simulink model "LabPSU_CPU01"  (R2026b)
undefined symbols (not defined in the file or in its folder): bit, Ctl_ipcTs, currentMeasured, enable, measurement, openLoopSetpoint, opmode, reference, slewrate, voltageMeasured
libraries: c2802xlib x2, procinterlib x2, c2000lib x1, c2837xDlib x1
settings Model: Creator=BenjaminRupp  LastModifiedBy=BenjaminRupp

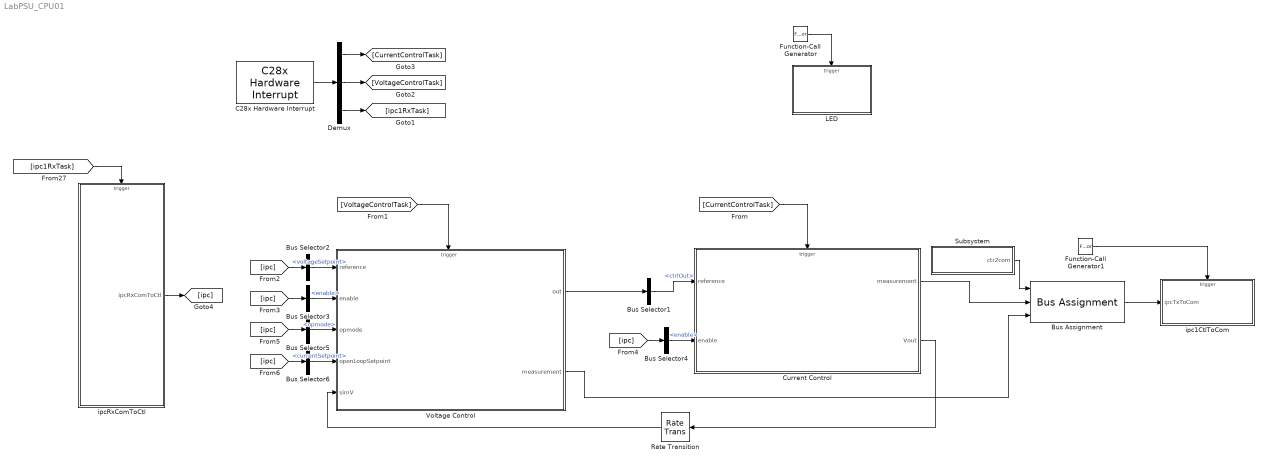
== system LabPSU_CPU01 ==
  Bus Assignment : BusAssignment  AssignedSignals=currentMeasured,voltageMeasured
  Bus Selector1 : BusSelector  OutputSignals=ctrlOut
  Bus Selector2 : BusSelector  OutputSignals=voltageSetpoint
  Bus Selector3 : BusSelector  OutputSignals=enable
  Bus Selector4 : BusSelector  OutputSignals=enable
  Bus Selector5 : BusSelector  OutputSignals=opmode
  Bus Selector6 : BusSelector  OutputSignals=currentSetpoint
  C28x Hardware Interrupt : c2000lib/Scheduling/C28x Hardware Interrupt  irqnumbers=[1 1 1]  pienumbers=[1 2 14]  irqpriorities=[30 29 28]  irqpreempts=[0 0 0]  showinput=off  dspchiptype=C280X
  Current Control : Subsystem
  Demux : Demux  Outputs=3
  Function-Call Generator : FunctionCallGenerator  SampleTime=0.1
  Function-Call Generator1 : FunctionCallGenerator  SampleTime=Ctl_ipcTs
  LED : Subsystem
  Rate Transition : RateTransition  Integrity=off
  Subsystem : Subsystem
  Voltage Control : Subsystem
  ipc1CtlToCom : Subsystem
  ipcRxComToCtl : Subsystem
  wires:
  Demux/1 -> [CurrentControlTask]
  Demux/3 -> [ipc1RxTask]
  C28x Hardware Interrupt/1 -> Demux/1
  Demux/2 -> [VoltageControlTask]
  Function-Call Generator/1 -> LED/Trigger
  [ipc1RxTask] -> ipcRxComToCtl/Trigger
  Function-Call Generator1/1 -> ipc1CtlToCom/Trigger
  [CurrentControlTask] -> Current Control/Trigger
  [VoltageControlTask] -> Voltage Control/Trigger
  Subsystem/1(ctr2com) -> Bus Assignment/1
  Bus Assignment/1 -> ipc1CtlToCom/1(ipcTxToCom)
  Current Control/1(measurement) -> Bus Assignment/2
  Voltage Control/2(measurement) -> Bus Assignment/3
  Voltage Control/1(out) -> Bus Selector1/1
  Bus Selector1/1 -> Current Control/1(reference)  "<ctrlOut>"
  ipcRxComToCtl/1(ipcRxComToCtl) -> [ipc]
  [ipc] -> Bus Selector2/1
  Bus Selector2/1 -> Voltage Control/1(reference)  "<voltageSetpoint>"
  Bus Selector3/1 -> Voltage Control/2(enable)  "<enable>"
  [ipc] -> Bus Selector3/1
  Bus Selector4/1 -> Current Control/2(enable)  "<enable>"
  [ipc] -> Bus Selector4/1
  [ipc] -> Bus Selector5/1
  Bus Selector5/1 -> Voltage Control/3(opmode)  "<opmode>"
  [ipc] -> Bus Selector6/1
  Bus Selector6/1 -> Voltage Control/4(openLoopSetpoint)  "<currentSetpoint>"
  Current Control/2(Vout) -> Rate Transition/1
  Rate Transition/1 -> Voltage Control/5(simV)

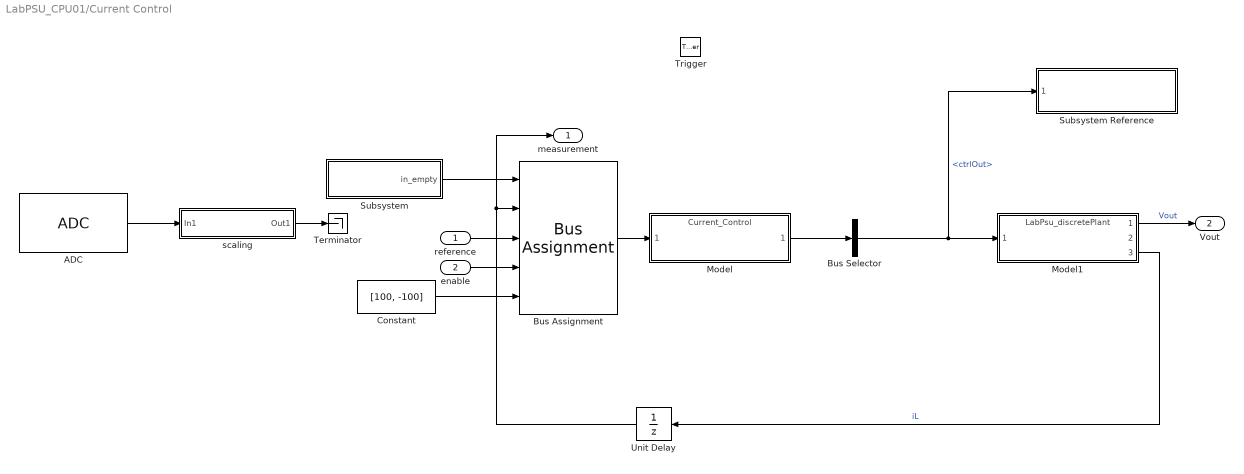
== system LabPSU_CPU01/Current Control ==
  reference : Inport  OutDataTypeStr=single
  enable : Inport  Port=2  OutDataTypeStr=uint16
  Trigger : TriggerPort  TriggerType=function-call  VariantControl=(inherit)  PortDimensions=1
  ADC : c2802xlib/ADC  blkParamProc=C2000_Type4  ADCModule=A  samplingMode=Single sample mode  ADCResolution=12-bit (Single-ended input)  ADC29xResolution=12-bit  ADCMode=Single-ended input  useSOC1=SOC0  useSOC2=SOC0_SOC1  SOCAcquisitionWindow=15  SOCTriggerSource=ePWM4_ADCSOCA  SOCInterruptTrigger=No ADCINT  Ts=-1  dType=single  postInterrupt=on  interruptSel=ADCINT1  ADCINTContinuous=on  endma=off  chdma=1  conv1=ADCINA0  conv2=ADCINA0 and ADCINB0  conv1_Type4=ADCIN0  conv2_Type4=ADCIN0 and ADCIN1
      settings: LibrarySourceBlock=c2837xDlib/ADC
  Bus Assignment : BusAssignment  AssignedSignals=measurement,reference,enable,slewrate
  Bus Selector : BusSelector  OutputSignals=ctrlOut
  Constant : Constant  Value=[100, -100]  OutDataTypeStr=single  SampleTime=-1
  Model : ModelReference  ModelNameDialog=Current_Control.slx  SimulationMode=Normal  ModelReferenceVersion=3.0
  Model1 : ModelReference  ModelNameDialog=LabPsu_discretePlant.slx  SimulationMode=Normal  ModelReferenceVersion=3.0
  Subsystem : Subsystem
  Subsystem Reference : Subsystem  ReferencedSubsystem=LabPsu_Pwm
  Terminator : Terminator
  Unit Delay : UnitDelay  SampleTime=-1
  scaling : Subsystem
  measurement : Outport
  Vout : Outport  Port=2
  wires:
  Bus Assignment/1 -> Model/1
  Model/1 -> Bus Selector/1
  Bus Selector/1 -> Model1/1, Subsystem Reference/1  "<ctrlOut>"
  Subsystem/1(in_empty) -> Bus Assignment/1
  ADC/1 -> scaling/1(In1)
  reference/1 -> Bus Assignment/3
  enable/1 -> Bus Assignment/4
  Constant/1 -> Bus Assignment/5
  Unit Delay/1 -> Bus Assignment/2, measurement/1
  Model1/3 -> Unit Delay/1  "iL"
  Model1/1 -> Vout/1  "Vout"
  scaling/1(Out1) -> Terminator/1

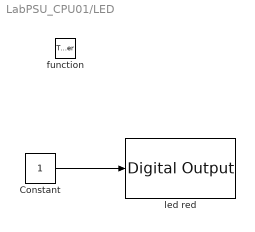
== system LabPSU_CPU01/LED ==
  function : TriggerPort  TriggerType=function-call  VariantControl=(inherit)
  Constant : Constant
  led red : c2837xDlib/Digital Output  GPIO_Number=GPIO24~GPIO31  GPIO_Bit0=off  GPIO_BIT0_Toggle=off  GPIO_Bit1=off  GPIO_BIT1_Toggle=off  GPIO_Bit2=off  GPIO_BIT2_Toggle=off  GPIO_Bit3=off  GPIO_BIT3_Toggle=off  GPIO_Bit4=off  GPIO_BIT4_Toggle=off  GPIO_Bit5=off  GPIO_BIT5_Toggle=off  GPIO_Bit6=off  GPIO_BIT6_Toggle=off  GPIO_Bit7=on  GPIO_BIT7_Toggle=on
  wires:
  Constant/1 -> led red/1

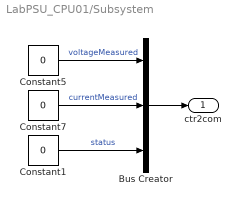
== system LabPSU_CPU01/Subsystem ==
  Bus Creator : BusCreator  Inputs=3  OutDataTypeStr=Bus: ctrl2com
  Constant1 : Constant  Value=0  OutDataTypeStr=uint16  SampleTime=-1
  Constant5 : Constant  Value=0  OutDataTypeStr=single  SampleTime=-1
  Constant7 : Constant  Value=0  OutDataTypeStr=single  SampleTime=-1
  ctr2com : Outport  OutDataTypeStr=Bus: ctrl2com
  wires:
  Bus Creator/1 -> ctr2com/1
  Constant5/1 -> Bus Creator/1  "voltageMeasured"
  Constant7/1 -> Bus Creator/2  "currentMeasured"
  Constant1/1 -> Bus Creator/3  "status"

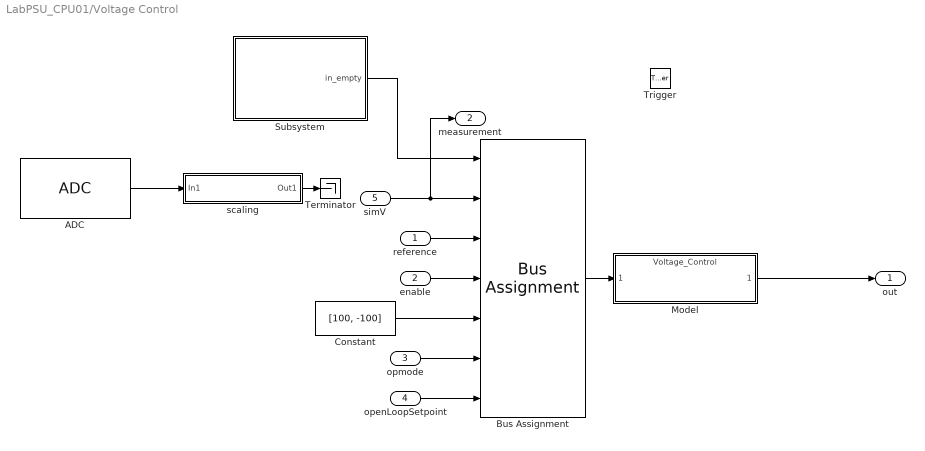
== system LabPSU_CPU01/Voltage Control ==
  reference : Inport  OutDataTypeStr=single
  enable : Inport  Port=2  OutDataTypeStr=uint16
  opmode : Inport  Port=3  OutDataTypeStr=uint16
  openLoopSetpoint : Inport  Port=4  OutDataTypeStr=single
  simV : Inport  Port=5
  Trigger : TriggerPort  TriggerType=function-call  VariantControl=(inherit)  PortDimensions=1
  ADC : c2802xlib/ADC  blkParamProc=C2000_Type4  ADCModule=B  samplingMode=Single sample mode  ADCResolution=12-bit (Single-ended input)  ADC29xResolution=12-bit  ADCMode=Single-ended input  useSOC1=SOC0  useSOC2=SOC0_SOC1  SOCAcquisitionWindow=15  SOCTriggerSource=ePWM5_ADCSOCA  SOCInterruptTrigger=No ADCINT  Ts=-1  dType=single  postInterrupt=on  interruptSel=ADCINT1  ADCINTContinuous=on  endma=off  chdma=1  conv1=ADCINA0  conv2=ADCINA0 and ADCINB0  conv1_Type4=ADCIN0  conv2_Type4=ADCIN0 and ADCIN1
      settings: LibrarySourceBlock=c2837xDlib/ADC
  Bus Assignment : BusAssignment  AssignedSignals=measurement,reference,enable,slewrate,opmode,openLoopSetpoint
  Constant : Constant  Value=[100, -100]  OutDataTypeStr=single  SampleTime=-1
  Model : ModelReference  ModelNameDialog=Voltage_Control.slx  SimulationMode=Normal  ModelReferenceVersion=3.0
  Subsystem : Subsystem
  Terminator : Terminator
  scaling : Subsystem
  out : Outport
  measurement : Outport  Port=2
  wires:
  Model/1 -> out/1
  ADC/1 -> scaling/1(In1)
  reference/1 -> Bus Assignment/3
  Constant/1 -> Bus Assignment/5
  enable/1 -> Bus Assignment/4
  Subsystem/1(in_empty) -> Bus Assignment/1
  Bus Assignment/1 -> Model/1
  simV/1 -> measurement/1, Bus Assignment/2
  opmode/1 -> Bus Assignment/6
  openLoopSetpoint/1 -> Bus Assignment/7
  scaling/1(Out1) -> Terminator/1

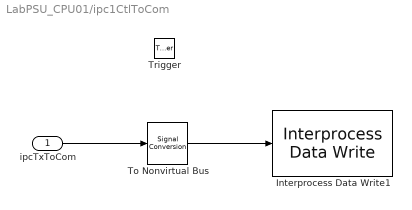
== system LabPSU_CPU01/ipc1CtlToCom ==
  ipcTxToCom : Inport  OutDataTypeStr=Bus: ctrl2com
  Trigger : TriggerPort  TriggerType=function-call  VariantControl=(inherit)  PortDimensions=1
  Interprocess Data Write1 : procinterlib/Interprocess Data Write  showPort=off  ChannelNum=6  NumBuff=1  IsIntEnabled=0  EnInterrupt=off  IPCBetween=0  CurrentPU=0  DataType=uint8  PartCores=CPU1<->CPU2  TargetType=0  ClientPU=TriCore1  ClientIntPrio=50  CurrentPUPriority=0  TargetName=0
      settings: LibrarySourceBlock=c2000lib/Target Communication/Interprocess Data Write
  To Nonvirtual Bus : SignalConversion  ConversionOutput=Nonvirtual bus  OverrideOpt=off
  wires:
  To Nonvirtual Bus/1 -> Interprocess Data Write1/1
  ipcTxToCom/1 -> To Nonvirtual Bus/1

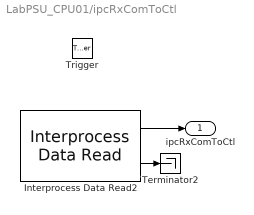
== system LabPSU_CPU01/ipcRxComToCtl ==
  Trigger : TriggerPort  TriggerType=function-call  VariantControl=(inherit)  PortDimensions=1
  Interprocess Data Read2 : procinterlib/Interprocess Data Read  Priority=3  showPort=off  DataType=Bus: com2ctrl  NumBuffers=1  DataLength=1  ChannelNum=1  IsIntEnabled=1  EnInterrupt=on  StructForBus=struct('voltageSetpoint',single(zeros(1,1)),'enable',uint16(zeros(1,1)),'opmode',uint16(zeros(1,1)),'currentSetpoint',single(zeros(1,1)))  IPCBetween=0  CurrentPU=0  PartCores=CPU1<->CPU2  SampleTime=-1  TargetType=0  ClientPU=TriCore1  ClientIntPrio=50  CurrentPUPriority=0  TargetName=0
      settings: LibrarySourceBlock=c2000lib/Target Communication/Interprocess Data Read
  Terminator2 : Terminator
  ipcRxComToCtl : Outport  OutDataTypeStr=Bus: com2ctrl
  wires:
  Interprocess Data Read2/2 -> Terminator2/1
  Interprocess Data Read2/1 -> ipcRxComToCtl/1

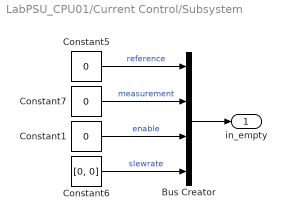
== system LabPSU_CPU01/Current Control/Subsystem ==
  Bus Creator : BusCreator  Inputs=4  OutDataTypeStr=Bus: CurrentControl_in
  Constant1 : Constant  Value=0  OutDataTypeStr=uint16  SampleTime=-1
  Constant5 : Constant  Value=0  OutDataTypeStr=single  SampleTime=-1
  Constant6 : Constant  Value=[0, 0]  OutDataTypeStr=single  SampleTime=-1
  Constant7 : Constant  Value=0  OutDataTypeStr=single  SampleTime=-1
  in_empty : Outport
  wires:
  Bus Creator/1 -> in_empty/1
  Constant5/1 -> Bus Creator/1  "reference"
  Constant6/1 -> Bus Creator/4  "slewrate"
  Constant7/1 -> Bus Creator/2  "measurement"
  Constant1/1 -> Bus Creator/3  "enable"

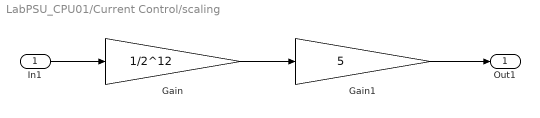
== system LabPSU_CPU01/Current Control/scaling ==
  In1 : Inport
  Gain : Gain  Gain=1/2^12
  Gain1 : Gain  Gain=5
  Out1 : Outport
  wires:
  Gain/1 -> Gain1/1
  In1/1 -> Gain/1
  Gain1/1 -> Out1/1

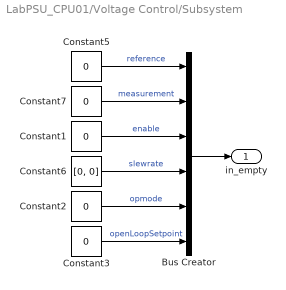
== system LabPSU_CPU01/Voltage Control/Subsystem ==
  Bus Creator : BusCreator  Inputs=6  OutDataTypeStr=Bus: VoltageControl_in
  Constant1 : Constant  Value=0  OutDataTypeStr=uint16  SampleTime=-1
  Constant2 : Constant  Value=0  OutDataTypeStr=uint16  SampleTime=-1
  Constant3 : Constant  Value=0  OutDataTypeStr=single  SampleTime=-1
  Constant5 : Constant  Value=0  OutDataTypeStr=single  SampleTime=-1
  Constant6 : Constant  Value=[0, 0]  OutDataTypeStr=single  SampleTime=-1
  Constant7 : Constant  Value=0  OutDataTypeStr=single  SampleTime=-1
  in_empty : Outport
  wires:
  Bus Creator/1 -> in_empty/1
  Constant5/1 -> Bus Creator/1  "reference"
  Constant6/1 -> Bus Creator/4  "slewrate"
  Constant7/1 -> Bus Creator/2  "measurement"
  Constant1/1 -> Bus Creator/3  "enable"
  Constant2/1 -> Bus Creator/5  "opmode"
  Constant3/1 -> Bus Creator/6  "openLoopSetpoint"

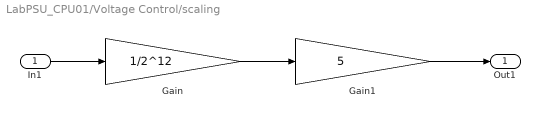
== system LabPSU_CPU01/Voltage Control/scaling ==
  In1 : Inport
  Gain : Gain  Gain=1/2^12
  Gain1 : Gain  Gain=5
  Out1 : Outport
  wires:
  Gain/1 -> Gain1/1
  In1/1 -> Gain/1
  Gain1/1 -> Out1/1
